simulink subsystem "smart_joystick"  (R2026a)
settings: Solver=VariableStepAuto
undefined symbols (not defined in the file): DiscIntNeverNeededParam, dspblkCoreblockFVToolHelper, FF_maneuvers, gcbh, I, P, S, T
libraries: slpidlib x3
settings Model: Creator=koryh  LastModifiedBy=kjhaydon

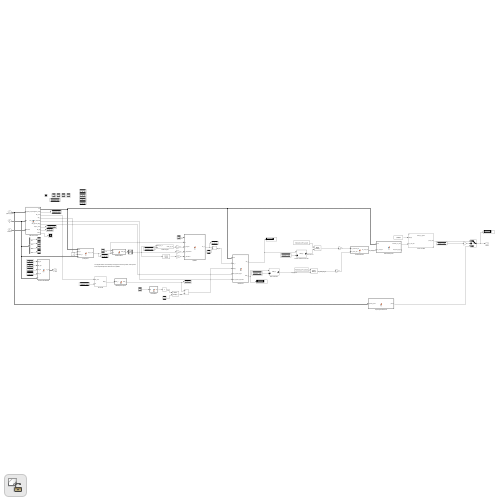
[thumbnail: Simulink's stored preview of the top-level diagram]
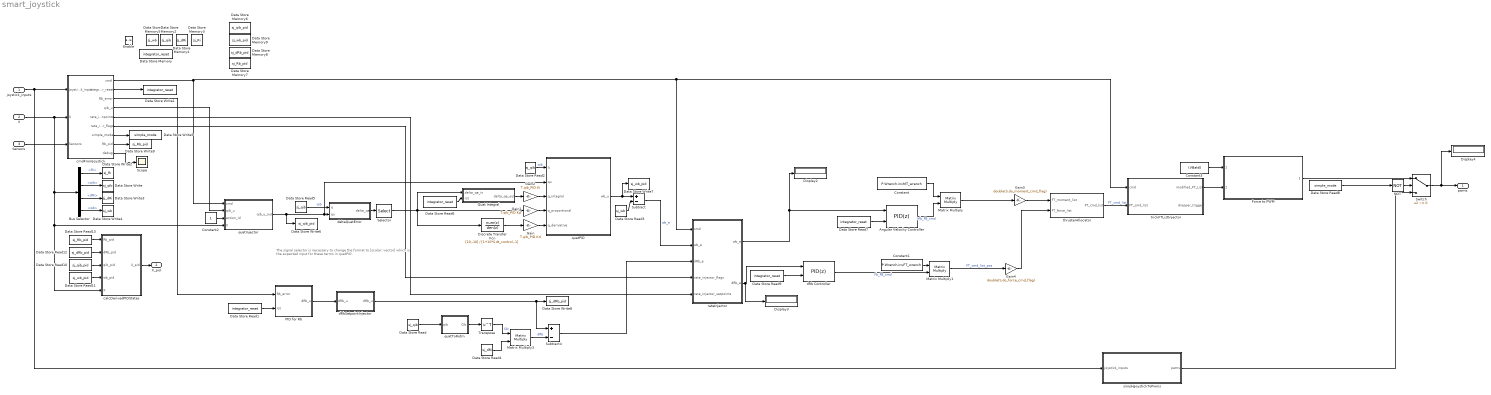
== system smart_joystick ==
  note: The signal selector is necessary to change the format to [scalar; vector] which
      | is the expected input for these terms in quatPID.
  joystick_inputs : Inport
  X : Inport  Port=2  SampleTime=S.dt_control
  Sensors : Inport  Port=3
  Enable : EnablePort
  Angular Velocity Controller : slpidlib/PID Controller  Controller=PID  Form=Parallel  TimeDomain=Discrete-time  UseExternalTs=off  SampleTime=-1  IntegratorMethod=Forward Euler  FilterMethod=Forward Euler  ControllerParametersSource=internal  P=T.wb_PID.Kp  I=T.wb_PID.Ki  UseKiTs=off  D=T.wb_PID.Kd  UseExternalDerivativeSource=off  N=T.wb_PID.N  UseFilter=on  TunerSelectOption=Transfer Function Based (PID Tuner App)  InitialConditionSource=internal  InitialConditionForIntegrator=0  InitialConditionForFilter=0  DifferentiatorICPrevScaledInput=0  ExternalReset=rising  TrackingMode=off  Kt=1  LimitOutput=on  SatLimitsSource=internal  UpperSaturationLimit=T.wb_PID.output_sat  LowerSaturationLimit=-T.wb_PID.output_sat  LinearizeAsGain=on  AntiWindupMode=clamping  Kb=1  LimitIntegrator=on  UpperIntegratorSaturationLimit=T.wb_PID.int_sat  LowerIntegratorSaturationLimit=-T.wb_PID.int_sat  POutMin=[]  POutMax=[]  IOutMin=[]  IOutMax=[]  DOutMin=[]  DOutMax=[]  NOutMin=[]  NOutMax=[]  SumOutMin=[]  SumOutMax=[]  SaturationOutMin=[]  SaturationOutMax=[]  PParamMin=[]  PParamMax=[]  IParamMin=[]  IParamMax=[]  DParamMin=[]  DParamMax=[]  NParamMin=[]  NParamMax=[]  KbParamMin=[]  KbParamMax=[]  KtParamMin=[]  KtParamMax=[]  KbOutMin=[]  KbOutMax=[]  KtOutMin=[]  KtOutMax=[]  IntegratorOutMin=[]  IntegratorOutMax=[]  FilterOutMin=[]  FilterOutMax=[]  SumI1OutMin=[]  SumI1OutMax=[]  SumI2OutMin=[]  SumI2OutMax=[]  SumI3OutMin=[]  SumI3OutMax=[]  SumI4OutMin=[]  SumI4OutMax=[]  SumDOutMin=[]  SumDOutMax=[]  DifferentiatorOutMin=[]  DifferentiatorOutMax=[]  FilterDiffOutCoefMin=[]  FilterDiffOutCoefMax=[]  ReciprocalOutMin=[]  ReciprocalOutMax=[]  SumDenOutMin=[]  SumDenOutMax=[]  SumNumOutMin=[]  SumNumOutMax=[]  DivideOutMin=[]  DivideOutMax=[]  UdiffTsProdOutMin=[]  UdiffTsProdOutMax=[]  NTsProdOutMin=[]  NTsProdOutMax=[]  UintegralTsProdOutMin=[]  UintegralTsProdOutMax=[]  UngainTsProdOutMin=[]  UngainTsProdOutMax=[]  ClampingZeroOutDataTypeStr=Inherit: Inherit via back propagation  ClampingZeroOutMin=[]  ClampingZeroOutMax=[]  FilterDenConstantOutDataTypeStr=Inherit: Inherit via back propagation  FilterDenConstantOutMin=[]  FilterDenConstantOutMax=[]  PCopyOutDataTypeStr=Inherit: Inherit via back propagation  PCopyOutMin=[]  PCopyOutMax=[]  NCopyOutDataTypeStr=Inherit: Inherit via back propagation  NCopyOutMin=[]  NCopyOutMax=[]  IntegratorContinuousStateAttributes=''  IntegratorStateMustResolveToSignalObject=off  IntegratorRTWStateStorageClass=Auto  FilterContinuousStateAttributes=''  FilterStateMustResolveToSignalObject=off  FilterRTWStateStorageClass=Auto  ParallelPVariant=InternalParameters  IdealPVariant=Disabled  IVariant=InternalParameters  DVariant=InternalParameters  IntegratorVariant=Discrete  SatVariant=Enabled  AWVariant=DiscClampingParallel  PCopyVariant=Disabled  TRVariant=Disabled  FdbkBlocksVariant=Forward  IdealPFdbkVariant=Disabled  SatFdbkVariant=Disabled  DerivativeFilterVariant=ForwardEulerFilter  NVariant=InternalParameters  NCopyVariant=Disabled  FilterICVariant=InternalICsFilter  IntegratorICVariant=InternalICs  ExternalResetVariant=ExternalReset  TRSumVariant=Passthrough  SumFdbkVariant=Disabled  SumVariant=Sum_PID  TsampFilterVariant=InternalTs  TsampNgainVariant=Passthrough  TsampIntegralVariant=Disabled_SignalSpec  ExternalSaturationOutDataTypeStr=Inherit: Same as second input  DerivativeSourceVariant=ErrorSignal  PreIntVariant=InternalPreInt
  Bus Selector : BusSelector  OutputSignals=Ri,qib,dRi,wb
  Constant : Constant  Value=P.Wrench.invMT_wrench
  Constant1 : Constant  Value=P.Wrench.invFT_wrench
  Constant2 : Constant
  Constant3 : Constant  Value=I.VBatt0
  Data Store Memory : DataStoreMemory  DataStoreName=integrator_reset  WriteAfterWriteMsg=warning  ShowAdditionalParam=off
  Data Store Memory2 : DataStoreMemory  DataStoreName=sj_qib  WriteAfterWriteMsg=warning  InitialValue=[0 0 0 1]'  ShowAdditionalParam=off
  Data Store Memory3 : DataStoreMemory  DataStoreName=sj_Ri  WriteAfterWriteMsg=warning  InitialValue=[0 0 0]'  ShowAdditionalParam=off
  Data Store Memory4 : DataStoreMemory  DataStoreName=sj_dRi  WriteAfterWriteMsg=warning  InitialValue=[0 0 0]'  ShowAdditionalParam=off
  Data Store Memory5 : DataStoreMemory  DataStoreName=sj_wb  WriteAfterWriteMsg=warning  InitialValue=[0 0 0]'  ShowAdditionalParam=off
  Data Store Memory6 : DataStoreMemory  DataStoreName=sj_qib_pid  WriteAfterWriteMsg=warning  InitialValue=[0 0 0 1]'  ShowAdditionalParam=off
  Data Store Memory7 : DataStoreMemory  DataStoreName=sj_Rb_pid  WriteAfterWriteMsg=warning  InitialValue=[0 0 0]'  ShowAdditionalParam=off
  Data Store Memory8 : DataStoreMemory  DataStoreName=sj_dRb_pid  WriteAfterWriteMsg=warning  InitialValue=[0 0 0]'  ShowAdditionalParam=off
  Data Store Memory9 : DataStoreMemory  DataStoreName=sj_wb_pid  WriteAfterWriteMsg=warning  InitialValue=[0 0 0]'  ShowAdditionalParam=off
  Data Store Read : DataStoreRead  DataStoreName=sj_qib  IndexOptions=Index vector (dialog)  Indices=1  OutputSizes=1
  Data Store Read{1,6..7,9} (4 alike) : DataStoreRead  DataStoreName=integrator_reset  IndexOptions=Index vector (dialog)  Indices=1  OutputSizes=1
  Data Store Read10 : DataStoreRead  DataStoreName=sj_qib_pid  IndexOptions=Index vector (dialog)  Indices=1  OutputSizes=1
  Data Store Read11 : DataStoreRead  DataStoreName=sj_wb_pid  IndexOptions=Index vector (dialog)  Indices=1  OutputSizes=1
  Data Store Read12 : DataStoreRead  DataStoreName=sj_dRb_pid  IndexOptions=Index vector (dialog)  Indices=1  OutputSizes=1
  Data Store Read13 : DataStoreRead  DataStoreName=sj_Rb_pid  IndexOptions=Index vector (dialog)  Indices=1  OutputSizes=1
  Data Store Read2 : DataStoreRead  DataStoreName=sj_qib  IndexOptions=Index vector (dialog)  Indices=1  OutputSizes=1
  Data Store Read3 : DataStoreRead  DataStoreName=sj_wb  IndexOptions=Index vector (dialog)  Indices=1  OutputSizes=1
  Data Store Read4 : DataStoreRead  DataStoreName=sj_dRi  IndexOptions=Index vector (dialog)  Indices=1  OutputSizes=1
  Data Store Read5 : DataStoreRead  DataStoreName=sj_qib  IndexOptions=Index vector (dialog)  Indices=1  OutputSizes=1
  Data Store Read8 : DataStoreRead  DataStoreName=simple_mode  IndexOptions=Index vector (dialog)  Indices=1  OutputSizes=1
  Data Store Write : DataStoreWrite  DataStoreName=sj_qib  IndexOptions=Index vector (dialog)  Indices=1  OutputSizes=1
  Data Store Write1 : DataStoreWrite  DataStoreName=integrator_reset  IndexOptions=Index vector (dialog)  Indices=1  OutputSizes=1
  Data Store Write2 : DataStoreWrite  DataStoreName=sj_Ri  IndexOptions=Index vector (dialog)  Indices=1  OutputSizes=1
  Data Store Write3 : DataStoreWrite  DataStoreName=sj_dRi  IndexOptions=Index vector (dialog)  Indices=1  OutputSizes=1
  Data Store Write4 : DataStoreWrite  DataStoreName=sj_wb  IndexOptions=Index vector (dialog)  Indices=1  OutputSizes=1
  Data Store Write5 : DataStoreWrite  DataStoreName=simple_mode  IndexOptions=Index vector (dialog)  Indices=1  OutputSizes=1
  Data Store Write6 : DataStoreWrite  DataStoreName=sj_qib_pid  IndexOptions=Index vector (dialog)  Indices=1  OutputSizes=1
  Data Store Write7 : DataStoreWrite  DataStoreName=sj_wb_pid  IndexOptions=Index vector (dialog)  Indices=1  OutputSizes=1
  Data Store Write8 : DataStoreWrite  DataStoreName=sj_dRb_pid  IndexOptions=Index vector (dialog)  Indices=1  OutputSizes=1
  Data Store Write9 : DataStoreWrite  DataStoreName=sj_Rb_pid  IndexOptions=Index vector (dialog)  Indices=1  OutputSizes=1
  Discrete Transfer Fcn : DiscreteTransferFcn  LoadFcn=dspblkCoreblockFVToolHelper(gcbh,'load');  Numerator=[10,-10]  Denominator=[1+10*S.dt_control,-1]
      settings: CopyFcn=dspblkCoreblockFVToolHelper(gcbh,'copy');  DeleteFcn=dspblkCoreblockFVToolHelper(gcbh,'close');  ModelCloseFcn=dspblkCoreblockFVToolHelper(gcbh,'close');  PreSaveFcn=dspblkCoreblockFVToolHelper(gcbh,'presave');  PostSaveFcn=dspblkCoreblockFVToolHelper(gcbh,'postsave');  CloseFcn=dspblkCoreblockFVToolHelper(gcbh,'close');
  Display2 : Display
  Display3 : Display
  Display4 : Display
  Force to PWM : Subsystem  ReferencedSubsystem=force_to_pwm
  Gain : Gain  Gain=T.qib_PID.Kd
  Gain1 : Gain  Gain=T.qib_PID.Kp
  Gain2 : Gain  Gain=T.qib_PID.Ki
  Gain3 : Gain  Gain=double(S.do_moment_cmd_flag)
  Gain4 : Gain  Gain=double(S.do_force_cmd_flag)
  Matrix Multiply : Product  Multiplication=Matrix(*)
  Matrix Multiply1 : Product  Multiplication=Matrix(*)
  Matrix Multiply3 : Product  Multiplication=Matrix(*)
  NOT : Logic  Operator=NOT  IconShape=distinctive  AllPortsSameDT=off  OutDataTypeStr=boolean
  PID for Rb : Subsystem
  Quat Integral : Subsystem
  Scope : Scope
      settings: ActiveDisplayYMinimum=-1  ActiveDisplayYMaximum=1
  Selector : Selector  InputPortWidth=4  IndexOptions=Index vector (dialog)  Indices=[4 1 2 3]  OutputSizes=1
  Subtract : Sum  Inputs=+-
  Subtract4 : Sum  Inputs=+-
  Switch : Switch  Criteria=u2 ~= 0  SaturateOnIntegerOverflow=off  InputSameDT=off
  Transpose : Math  Operator=transpose
  calcDerivedPIDStates : MATLAB Function  TreatAsAtomicUnit=on
  cmdFromJoystick : MATLAB Function  TreatAsAtomicUnit=on
  dRb Controller : slpidlib/PID Controller  Controller=PID  Form=Parallel  TimeDomain=Discrete-time  UseExternalTs=off  SampleTime=-1  IntegratorMethod=Forward Euler  FilterMethod=Forward Euler  ControllerParametersSource=internal  P=T.dRb_PID.Kp  I=T.dRb_PID.Ki  UseKiTs=off  D=T.dRb_PID.Kd  UseExternalDerivativeSource=off  N=T.dRb_PID.N  UseFilter=on  TunerSelectOption=Transfer Function Based (PID Tuner App)  InitialConditionSource=internal  InitialConditionForIntegrator=0  InitialConditionForFilter=0  DifferentiatorICPrevScaledInput=0  ExternalReset=rising  TrackingMode=off  Kt=1  LimitOutput=on  SatLimitsSource=internal  UpperSaturationLimit=T.dRb_PID.output_sat  LowerSaturationLimit=-T.dRb_PID.output_sat  LinearizeAsGain=on  AntiWindupMode=clamping  Kb=1  LimitIntegrator=on  UpperIntegratorSaturationLimit=T.dRb_PID.int_sat  LowerIntegratorSaturationLimit=-T.dRb_PID.int_sat  POutMin=[]  POutMax=[]  IOutMin=[]  IOutMax=[]  DOutMin=[]  DOutMax=[]  NOutMin=[]  NOutMax=[]  SumOutMin=[]  SumOutMax=[]  SaturationOutMin=[]  SaturationOutMax=[]  PParamMin=[]  PParamMax=[]  IParamMin=[]  IParamMax=[]  DParamMin=[]  DParamMax=[]  NParamMin=[]  NParamMax=[]  KbParamMin=[]  KbParamMax=[]  KtParamMin=[]  KtParamMax=[]  KbOutMin=[]  KbOutMax=[]  KtOutMin=[]  KtOutMax=[]  IntegratorOutMin=[]  IntegratorOutMax=[]  FilterOutMin=[]  FilterOutMax=[]  SumI1OutMin=[]  SumI1OutMax=[]  SumI2OutMin=[]  SumI2OutMax=[]  SumI3OutMin=[]  SumI3OutMax=[]  SumI4OutMin=[]  SumI4OutMax=[]  SumDOutMin=[]  SumDOutMax=[]  DifferentiatorOutMin=[]  DifferentiatorOutMax=[]  FilterDiffOutCoefMin=[]  FilterDiffOutCoefMax=[]  ReciprocalOutMin=[]  ReciprocalOutMax=[]  SumDenOutMin=[]  SumDenOutMax=[]  SumNumOutMin=[]  SumNumOutMax=[]  DivideOutMin=[]  DivideOutMax=[]  UdiffTsProdOutMin=[]  UdiffTsProdOutMax=[]  NTsProdOutMin=[]  NTsProdOutMax=[]  UintegralTsProdOutMin=[]  UintegralTsProdOutMax=[]  UngainTsProdOutMin=[]  UngainTsProdOutMax=[]  ClampingZeroOutDataTypeStr=Inherit: Inherit via back propagation  ClampingZeroOutMin=[]  ClampingZeroOutMax=[]  FilterDenConstantOutDataTypeStr=Inherit: Inherit via back propagation  FilterDenConstantOutMin=[]  FilterDenConstantOutMax=[]  PCopyOutDataTypeStr=Inherit: Inherit via back propagation  PCopyOutMin=[]  PCopyOutMax=[]  NCopyOutDataTypeStr=Inherit: Inherit via back propagation  NCopyOutMin=[]  NCopyOutMax=[]  IntegratorContinuousStateAttributes=''  IntegratorStateMustResolveToSignalObject=off  IntegratorRTWStateStorageClass=Auto  FilterContinuousStateAttributes=''  FilterStateMustResolveToSignalObject=off  FilterRTWStateStorageClass=Auto  ParallelPVariant=InternalParameters  IdealPVariant=Disabled  IVariant=InternalParameters  DVariant=InternalParameters  IntegratorVariant=Discrete  SatVariant=Enabled  AWVariant=DiscClampingParallel  PCopyVariant=Disabled  TRVariant=Disabled  FdbkBlocksVariant=Forward  IdealPFdbkVariant=Disabled  SatFdbkVariant=Disabled  DerivativeFilterVariant=ForwardEulerFilter  NVariant=InternalParameters  NCopyVariant=Disabled  FilterICVariant=InternalICsFilter  IntegratorICVariant=InternalICs  ExternalResetVariant=ExternalReset  TRSumVariant=Passthrough  SumFdbkVariant=Disabled  SumVariant=Sum_PID  TsampFilterVariant=InternalTs  TsampNgainVariant=Passthrough  TsampIntegralVariant=Disabled_SignalSpec  ExternalSaturationOutDataTypeStr=Inherit: Same as second input  DerivativeSourceVariant=ErrorSignal  PreIntVariant=InternalPreInt
  dRbSetpointInjector : MATLAB Function  TreatAsAtomicUnit=on
  deltaQuatError : MATLAB Function  TreatAsAtomicUnit=on
  quatInjector : MATLAB Function  TreatAsAtomicUnit=on
  quatPID : MATLAB Function  TreatAsAtomicUnit=on
  quatToRotm : MATLAB Function  TreatAsAtomicUnit=on
  rateInjector : MATLAB Function  TreatAsAtomicUnit=on
  simpleJoystickToPwms : MATLAB Function  TreatAsAtomicUnit=on
  thrusterAllocator : MATLAB Function  TreatAsAtomicUnit=on
  trickFTListInjector : MATLAB Function  TreatAsAtomicUnit=on
  pwms : Outport
  X_pid : Outport  Port=2
  wires:
  cmdFromJoystick/1(cmd) -> quatInjector/1(cmd), trickFTListInjector/1(cmd), rateInjector/1(cmd)
  quatToRotm/1(Cib) -> Transpose/1
  thrusterAllocator/1(FT_cmd_list) -> trickFTListInjector/2(FT_cmd_list)  "FT_cmd_list"
  Selector/1 -> Discrete Transfer Fcn/1, Quat Integral/1(delta_qe_in), Gain1/1
  Data Store Read9/1 -> dRb Controller/2
  Data Store Read7/1 -> Angular Velocity Controller/2
  Bus Selector/2 -> Data Store Write/1  "<qib>"
  Data Store Read2/1 -> quatPID/1(q)  "qib"
  quatPID/1(wb_u) -> Subtract/1, Data Store Write7/1
  Constant1/1 -> Matrix Multiply1/1
  Data Store Read3/1 -> Subtract/2
  Bus Selector/4 -> Data Store Write4/1  "<wb>"
  Data Store Read1/1 -> PID for Rb/2(rst)
  Gain2/1 -> quatPID/3(q_integral)
  Bus Selector/1 -> Data Store Write2/1  "<Ri>"
  Discrete Transfer Fcn/1 -> Gain/1
  dRbSetpointInjector/1(dRb_u) -> Subtract4/1, Data Store Write8/1
  rateInjector/1(wb_e) -> Angular Velocity Controller/1, Display2/1
  deltaQuatError/1(delta_qe) -> Selector/1
  Constant3/1 -> Force to PWM/1
  Constant/1 -> Matrix Multiply/1
  Transpose/1 -> Matrix Multiply3/1  "Cbi"
  Data Store Read5/1 -> deltaQuatError/1(q)  "qib"
  Subtract4/1 -> rateInjector/3("dRb_e ")
  Gain/1 -> quatPID/5(q_derivative)
  Matrix Multiply3/1 -> Subtract4/2  "dRb"
  trickFTListInjector/1(modified_FT_List) -> Force to PWM/2
  quatInjector/1(qib_u_out) -> Data Store Write6/1, quatPID/2(qu), deltaQuatError/2(qu)
  PID for Rb/1(dRb_u) -> dRbSetpointInjector/1("dRb_u ")
  Data Store Read6/1 -> Quat Integral/2(rst)
  Gain1/1 -> quatPID/4(q_proportional)
  rateInjector/2(dRb_e) -> dRb Controller/1, Display3/1
  Data Store Read4/1 -> Matrix Multiply3/2
  Data Store Read/1 -> quatToRotm/1(qib)
  Subtract/1 -> rateInjector/2("wb_e ")  "wb_e"
  Bus Selector/3 -> Data Store Write3/1  "<dRi>"
  Quat Integral/1(delta_qe_out) -> Gain2/1
  X/1 -> cmdFromJoystick/2(X), quatInjector/4(X), calcDerivedPIDStates/5(X), Bus Selector/1
  cmdFromJoystick/2(integrator_reset) -> Data Store Write1/1
  cmdFromJoystick/3(Rb_error) -> PID for Rb/1(Rb_error)
  cmdFromJoystick/4(qib_u) -> quatInjector/2(qib_u)
  Constant2/1 -> quatInjector/3(action_id)
  cmdFromJoystick/5(rate_injector_setpoints) -> rateInjector/5(rate_injector_setpoints)
  cmdFromJoystick/6(rate_injector_flags) -> rateInjector/4(rate_injector_flags)
  Sensors/1 -> cmdFromJoystick/3(Sensors)
  cmdFromJoystick/8(Rb_pid) -> Data Store Write9/1
  cmdFromJoystick/7(simple_mode) -> Data Store Write5/1
  joystick_inputs/1 -> cmdFromJoystick/1(joystick_input), simpleJoystickToPwms/1(joystick_inputs)
  Switch/1 -> pwms/1, Display4/1
  Force to PWM/1 -> Switch/1
  simpleJoystickToPwms/1(pwms) -> Switch/3
  Data Store Read8/1 -> NOT/1
  Data Store Read10/1 -> calcDerivedPIDStates/3(qib_pid)
  Data Store Read12/1 -> calcDerivedPIDStates/2(dRb_pid)
  Data Store Read11/1 -> calcDerivedPIDStates/4(wb_pid)
  Data Store Read13/1 -> calcDerivedPIDStates/1(Rb_pid)
  calcDerivedPIDStates/1(X_pid) -> X_pid/1
  NOT/1 -> Switch/2
  cmdFromJoystick/9(debug) -> Scope/1
  Matrix Multiply1/1 -> Gain4/1  "FT_cmd_list_pos"
  Gain4/1 -> thrusterAllocator/2(FT_force_list)
  Gain3/1 -> thrusterAllocator/1(FT_moment_list)
  Matrix Multiply/1 -> Gain3/1
  Angular Velocity Controller/1 -> Matrix Multiply/2  "Mb_FB_cmd"
  dRb Controller/1 -> Matrix Multiply1/2  "Fb_FB_cmd"

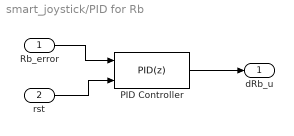
== system smart_joystick/PID for Rb ==
  Rb_error : Inport
  rst : Inport  Port=2
  PID Controller : slpidlib/PID Controller  Controller=PID  Form=Parallel  TimeDomain=Discrete-time  UseExternalTs=off  SampleTime=-1  IntegratorMethod=Forward Euler  FilterMethod=Forward Euler  ControllerParametersSource=internal  P=T.Rb_PID.Kp  I=T.Rb_PID.Ki  UseKiTs=off  D=T.Rb_PID.Kd  UseExternalDerivativeSource=off  N=T.Rb_PID.N  UseFilter=on  TunerSelectOption=Transfer Function Based (PID Tuner App)  InitialConditionSource=internal  InitialConditionForIntegrator=0  InitialConditionForFilter=0  DifferentiatorICPrevScaledInput=0  ExternalReset=rising  TrackingMode=off  Kt=1  LimitOutput=on  SatLimitsSource=internal  UpperSaturationLimit=T.Rb_PID.output_sat  LowerSaturationLimit=-T.Rb_PID.output_sat  LinearizeAsGain=on  AntiWindupMode=clamping  Kb=1  LimitIntegrator=on  UpperIntegratorSaturationLimit=T.Rb_PID.int_sat  LowerIntegratorSaturationLimit=-T.Rb_PID.int_sat  POutMin=[]  POutMax=[]  IOutMin=[]  IOutMax=[]  DOutMin=[]  DOutMax=[]  NOutMin=[]  NOutMax=[]  SumOutMin=[]  SumOutMax=[]  SaturationOutMin=[]  SaturationOutMax=[]  PParamMin=[]  PParamMax=[]  IParamMin=[]  IParamMax=[]  DParamMin=[]  DParamMax=[]  NParamMin=[]  NParamMax=[]  KbParamMin=[]  KbParamMax=[]  KtParamMin=[]  KtParamMax=[]  KbOutMin=[]  KbOutMax=[]  KtOutMin=[]  KtOutMax=[]  IntegratorOutMin=[]  IntegratorOutMax=[]  FilterOutMin=[]  FilterOutMax=[]  SumI1OutMin=[]  SumI1OutMax=[]  SumI2OutMin=[]  SumI2OutMax=[]  SumI3OutMin=[]  SumI3OutMax=[]  SumI4OutMin=[]  SumI4OutMax=[]  SumDOutMin=[]  SumDOutMax=[]  DifferentiatorOutMin=[]  DifferentiatorOutMax=[]  FilterDiffOutCoefMin=[]  FilterDiffOutCoefMax=[]  ReciprocalOutMin=[]  ReciprocalOutMax=[]  SumDenOutMin=[]  SumDenOutMax=[]  SumNumOutMin=[]  SumNumOutMax=[]  DivideOutMin=[]  DivideOutMax=[]  UdiffTsProdOutMin=[]  UdiffTsProdOutMax=[]  NTsProdOutMin=[]  NTsProdOutMax=[]  UintegralTsProdOutMin=[]  UintegralTsProdOutMax=[]  UngainTsProdOutMin=[]  UngainTsProdOutMax=[]  ClampingZeroOutDataTypeStr=Inherit: Inherit via back propagation  ClampingZeroOutMin=[]  ClampingZeroOutMax=[]  FilterDenConstantOutDataTypeStr=Inherit: Inherit via back propagation  FilterDenConstantOutMin=[]  FilterDenConstantOutMax=[]  PCopyOutDataTypeStr=Inherit: Inherit via back propagation  PCopyOutMin=[]  PCopyOutMax=[]  NCopyOutDataTypeStr=Inherit: Inherit via back propagation  NCopyOutMin=[]  NCopyOutMax=[]  IntegratorContinuousStateAttributes=''  IntegratorStateMustResolveToSignalObject=off  IntegratorRTWStateStorageClass=Auto  FilterContinuousStateAttributes=''  FilterStateMustResolveToSignalObject=off  FilterRTWStateStorageClass=Auto  ParallelPVariant=InternalParameters  IdealPVariant=Disabled  IVariant=InternalParameters  DVariant=InternalParameters  IntegratorVariant=Discrete  SatVariant=Enabled  AWVariant=DiscClampingParallel  PCopyVariant=Disabled  TRVariant=Disabled  FdbkBlocksVariant=Forward  IdealPFdbkVariant=Disabled  SatFdbkVariant=Disabled  DerivativeFilterVariant=ForwardEulerFilter  NVariant=InternalParameters  NCopyVariant=Disabled  FilterICVariant=InternalICsFilter  IntegratorICVariant=InternalICs  ExternalResetVariant=ExternalReset  TRSumVariant=Passthrough  SumFdbkVariant=Disabled  SumVariant=Sum_PID  TsampFilterVariant=InternalTs  TsampNgainVariant=Passthrough  TsampIntegralVariant=Disabled_SignalSpec  ExternalSaturationOutDataTypeStr=Inherit: Same as second input  DerivativeSourceVariant=ErrorSignal  PreIntVariant=InternalPreInt
  dRb_u : Outport
  wires:
  rst/1 -> PID Controller/2
  PID Controller/1 -> dRb_u/1
  Rb_error/1 -> PID Controller/1

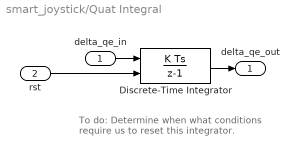
== system smart_joystick/Quat Integral ==
  note: To do: Determine when what conditions
      | require us to reset this integrator.
  delta_qe_in : Inport
  rst : Inport  Port=2
  Discrete-Time Integrator : DiscreteIntegrator  ExternalReset=rising  SampleTime=-1  LimitOutput=on  UpperSaturationLimit=T.qib_PID.int_sat  LowerSaturationLimit=-T.qib_PID.int_sat  ICPrevOutput=DiscIntNeverNeededParam  ICPrevScaledInput=DiscIntNeverNeededParam
  delta_qe_out : Outport
  wires:
  rst/1 -> Discrete-Time Integrator/2
  Discrete-Time Integrator/1 -> delta_qe_out/1
  delta_qe_in/1 -> Discrete-Time Integrator/1

== matlab function smart_joystick/quatPID ==
  data: q input; qu input; q_integral input; q_proportional input; wb_u output; q_derivative input; S parameter
function wb_u = fcn(q, qu, q_integral, q_proportional, q_derivative, S)

overwrite_rate_setpoint_flag = S.overwrite_rate_setpoint_flag;
wb_sp_inject = S.wb_sp_inject;

wb_u = quatPID(q, qu, q_proportional, q_integral, q_derivative, overwrite_rate_setpoint_flag, wb_sp_inject);

== matlab function smart_joystick/quatToRotm ==
  data: qib input; Cib output
function Cib = fcn(qib)

Cib = quatToRotm(qib);

== matlab function smart_joystick/thrusterAllocator ==
  data: FT_moment_list input; FT_cmd_list output; FT_force_list input; P parameter
function FT_cmd_list = fcn(FT_moment_list, FT_force_list, P)

max_thruster_force = P.Constants.max_thruster_force;

FT_cmd_list = thrusterAllocator(FT_moment_list, FT_force_list, max_thruster_force);

== matlab function smart_joystick/simpleJoystickToPwms ==
  data: pwms output size=[8 1]; joystick_inputs input Bus: joystick_bus
function pwms = fcn(joystick_inputs)

%Create the mapping here for PWM values.
%Recall that PWM 1-8 correspond to thruster postions which follow,

%pwm of each thruster on the robot
%In left to right:
%f = front / r = rear
%l = left  / r = right
%t = top   / b = bottom
%PWM(1)=pwm_flt
%PWM(2)=pwm_frt
%PWM(3)=pwm_rlt
%PWM(4)=pwm_rrt
%PWM(5)=pwm_flb
%PWM(6)=pwm_frb
%PWM(7)=pwm_rlb
%PWM(8)=pwm_rrb
  
x_joy = joystick_inputs.x;
y_joy = joystick_inputs.y;
rise = joystick_inputs.rise;
sink = joystick_inputs.sink;
yaw = joystick_inputs.yaw;
pitch = joystick_inputs.pitch;


scale = 200;
stop_set = 1500;
max_pwm = 1500+scale;
min_pwm = 1500-scale;

%x_body and y_body mapping
x = x_joy;
y = y_joy;

pwms_vert = stop_set*ones(1,4); %Thrusters 0,1,2,3
pwms_horiz = stop_set*ones(1,4); %Thrusters 4,5,6,7
inversion_mask = [1, -1, 1, -1];

% Rise/Sink
for i = 1:4
    pwms_vert(i) = pwms_vert(i) + (scale*rise - scale*sink) * inversion_mask(i);
end

%Pitch
pwms_vert(1) = pwms_vert(1) - (scale*pitch*inversion_mask(1));
pwms_vert(2) = pwms_vert(2) - (scale*pitch*inversion_mask(2));
pwms_vert(3) = pwms_vert(3) + (scale*pitch*inversion_mask(3));
pwms_vert(4) = pwms_vert(4) + (scale*pitch*inversion_mask(4));

% Forwards:
pwms_horiz(1) = pwms_horiz(1) + scale*x;
pwms_horiz(2) = pwms_horiz(2) - scale*x;
pwms_horiz(3) = pwms_horiz(3) + scale*x;
pwms_horiz(4) = pwms_horiz(4) - scale*x;

% Strafe:
pwms_horiz(1) = pwms_horiz(1) + y*scale;
pwms_horiz(2) = pwms_horiz(2) + y*scale;
pwms_horiz(3) = pwms_horiz(3) - y*scale;
pwms_horiz(4) = pwms_horiz(4) - y*scale;

% Yaw:
pwms_horiz(1) = pwms_horiz(1) + yaw*scale;
pwms_horiz(2) = pwms_horiz(2) + yaw*scale;
pwms_horiz(3) = pwms_horiz(3) + yaw*scale;
pwms_horiz(4) = pwms_horiz(4) + yaw*scale;


for i = 1:4
    if(pwms_horiz(i) > max_pwm)
        pwms_horiz(i) = max_pwm;
    end
    if(pwms_horiz(i) < min_pwm)
        pwms_horiz(i) = min_pwm;
    end
    if(pwms_vert(i) > max_pwm)
        pwms_vert(i) = max_pwm;
    end
    if(pwms_vert(i) < min_pwm)
        pwms_horiz(i) = min_pwm;
    end

end

pwms = [pwms_vert,pwms_horiz];
pwms = pwms(:);

== matlab function smart_joystick/deltaQuatError ==
  data: q input; delta_qe output; qu input; S parameter
function delta_qe = fcn(q, qu, S)

overwrite_state_error_flag = S.overwrite_state_error_flag;
eul_error_inject = S.eul_error_inject;

delta_qe = deltaQuatError(q, qu, overwrite_state_error_flag, eul_error_inject);

== matlab function smart_joystick/trickFTListInjector ==
  data: cmd input; modified_FT_List output size=[8,1]; FT_cmd_list input; FF_maneuvers parameter Bus: FF_maneuvers_bus; S parameter; dropper_trigger output
function [modified_FT_List, dropper_trigger] = fcn(cmd, FT_cmd_list, FF_maneuvers,S)

overwrite_FT_list_flag = S.overwrite_FT_list_flag;
FT_list_inject = S.FT_list_inject;

[modified_FT_List, dropper_trigger] = trickFTListInjector(cmd, FT_cmd_list, FF_maneuvers, overwrite_FT_list_flag, FT_list_inject);

== matlab function smart_joystick/cmdFromJoystick ==
  data: joystick_input input Bus: joystick_bus; cmd output Bus: cmd_bus; X input Bus: X_bus; integrator_reset output; Rb_error output; qib_u output; rate_injector_setpoints output; rate_injector_flags output; simple_mode output; T parameter; Sensors input; Rb_pid output; S parameter; debug output
function [cmd, integrator_reset, Rb_error, qib_u, rate_injector_setpoints, rate_injector_flags, simple_mode, Rb_pid, debug] = fcn(joystick_input, X, T, Sensors, S)

wb_tuning = T.js_wb_scale;
dRb_tuning = T.js_dRb_scale;
initial_simple_mode_flag = S.initial_simple_joystick_flag;

[cmd, integrator_reset, Rb_error, qib_u, rate_injector_setpoints, rate_injector_flags, simple_mode, Rb_pid, debug]...
    = cmdFromJoystick(joystick_input, X, wb_tuning, dRb_tuning, Sensors, initial_simple_mode_flag);

== matlab function smart_joystick/dRbSetpointInjector ==
  data: dRb_u input; dRb_u output; S parameter
function dRb_u=fcn(dRb_u, S)

dRb_sp_inject = S.dRb_sp_inject;
overwrite_rate_setpoint_flag = S.overwrite_rate_setpoint_flag;

if(overwrite_rate_setpoint_flag)
    dRb_u = dRb_sp_inject;
end

== matlab function smart_joystick/rateInjector ==
  data: cmd input Bus: cmd_bus; wb_e input; wb_e output; dRb_e input; dRb_e output; rate_injector_flags input; rate_injector_setpoints input
function [wb_e, dRb_e] = fcn(cmd, wb_e, dRb_e, rate_injector_flags, rate_injector_setpoints)

wb_error_inject = rate_injector_setpoints(4:6);
dRb_error_inject = rate_injector_setpoints(1:3);

[wb_e, dRb_e] = joystickRateInjector(cmd, wb_e, dRb_e, rate_injector_flags, wb_error_inject, dRb_error_inject);

== matlab function smart_joystick/calcDerivedPIDStates ==
  data: Rb_pid input; X_pid output Bus: X_bus; dRb_pid input; qib_pid input; wb_pid input; X input Bus: X_bus
function X_pid = fcn(Rb_pid, dRb_pid, qib_pid, wb_pid, X)

X_pid = calcDerivedPIDStates(Rb_pid, dRb_pid, qib_pid, wb_pid, X);

== matlab function smart_joystick/quatInjector ==
  data: cmd input; qib_u_out output size=[4 1]; qib_u input; action_id input; X input; S parameter
function qib_u_out  = fcn(cmd, qib_u, action_id, X, S)

eul_sp_inject = S.eul_sp_inject;
overwrite_state_setpoint_flag = S.overwrite_state_setpoint_flag;

qib_u_out = quatInjector(cmd, qib_u, action_id, X, eul_sp_inject, overwrite_state_setpoint_flag);
